simulink model "interleaved_boost"  (R2026b)
settings: Solver=ode23tb  StopTime=param.sim.simlength  FixedStep=tc  MaxStep=param.glb_time.tc
values from neighbouring files (symbols this model uses):
  param = struct()    [init_model.m]
libraries: fl_lib x138, nesl_utility x71, igbt_simple_2th_lib x6, single_phase_pwm_modulator x3, lithium_ion_battery x1, dclink_for_two_levels x1
(part 1 of 3)
settings Model: Creator=dbagn  LastModifiedBy=d.bagnara
settings SolverCC: SolverResetMethod=Robust  ZeroCrossControl=DisableAll
settings DataIOCC: DSMLogging=off  ReturnWorkspaceOutputs=off  SaveOutput=off  SaveTime=off  SignalLogging=off
settings OptimizationCC: ReuseModelBlockBuffer=off
settings SFSimCC: CustomCodeUndefinedFunction=ThrowError  DefaultCustomCodeDeterministicFunctions=All
settings SFSimCC: SimCustomHeaderCode=|
  | #include "rpi.h"
  | #include "rpi_simulink.h"
  | #include "bemf_obsv_load_est.h"
  | #include "bemf_obsv_load_est_simulink.h"
  | #include "dqpll_grid.h"
  | #include "dsmavgflt.h"
  | #include "bemf_obsv.h"
  | #include "bemf_obsv_simulink.h"
  | #include "mavgflt.h"
  | #include "mavgflt_simulink.h"
  | #include "mavgflts.h"
  | #include "mavgflts_simulink.h"
  | #include "sv_pwm_cm.h"
  | #include "dsmavgflt_simulink.h"
  | #include "linear_double_integrator_observer_simulink.h"
  | #include "sv_pwm_cm_simulink.h"
  | #include "dqvector_pi.h"
  | #include "dqpll_grid_simulink.h"
  | #include "first_harmonic_tracker.h"
  | #include "dqvector_pi_simulink.h"
  | #include "first_harmonic_tracker_simulink.h"
  | #include "dqpll_thyr.h"
  | #include "sv_pwm_simulink.h"
  | #include "sv_pwm.h"
  | #include "dqpll_thyr_simulink.h"
  | #include "linear_double_integrator_observer.h"
  | #include "math_f.h"
settings SFSimCC: SimUserIncludeDirs=|
  | include
  | src
settings SFSimCC: SimUserSources=|
  | "rpi.c"
  | "rpi_simulink.c"
  | "mavgflt_simulink.c"
  | "mavgflt.c"
  | "mavgflts_simulink.c"
  | "mavgflts.c"
  | "dsmavgflt_simulink.c"
  | "dsmavgflt.c"
  | "bemf_obsv_simulink.c"
  | "bemf_obsv.c"
  | "bemf_obsv_load_est_simulink.c"
  | "bemf_obsv_load_est.c"
  | "dqvector_pi.c"
  | "dqvector_pi_simulink.c"
  | "sv_pwm_simulink.c"
  | "sv_pwm.c"
  | "first_harmonic_tracker_simulink.c"
  | "first_harmonic_tracker.c"
  | "dqpll_thyr_simulink.c"
  | "dqpll_thyr.c"
  | "dqpll_grid_simulink.c"
  | "dqpll_grid.c"
  | "linear_double_integrator_observer_simulink.c"
  | "linear_double_integrator_observer.c"
  | "sv_pwm_cm_simulink.c"
  | "sv_pwm_cm.c"
settings RTWCC: DLArmComputeVersion=19.05
settings SimscapeCC: SimscapeUseEnergyAccounting=off

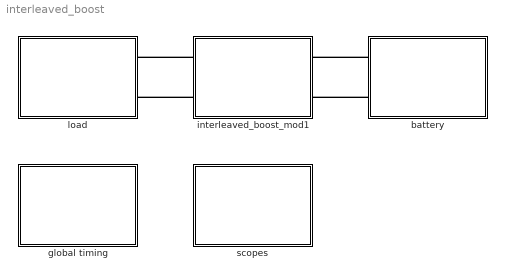
== system interleaved_boost ==
  battery : Subsystem
  global timing : Subsystem
  interleaved_boost_mod1 : Subsystem
  load : Subsystem
  scopes : Subsystem
  connections:
  interleaved_boost_mod1/RConn1 -- load/RConn1
  interleaved_boost_mod1/RConn2 -- load/RConn2
  battery/RConn2 -- interleaved_boost_mod1/LConn2
  battery/RConn1 -- interleaved_boost_mod1/LConn1

== system interleaved_boost/battery ==
  Electrical Reference : fl_lib/Electrical/Electrical Elements/Electrical Reference
  Solver Configuration : nesl_utility/Solver Configuration  PhysicalDomain=network_engine_domain  SubClassName=solver  LeftPortType=input  RightPortType=generic  Tones=[]  Harmonics=[]  SimulateNoise=off  Profile=off  UseLocalSampling=off  EnableSwitchedLinearOptims=on  FrequencyDomain=off  UseCCode=off  RelTol=0.001  AbsTol=0.001  MinStep=1e-09  ToWorkspace=off  RevertToSquareIcSolve=off  NumHomotopyIterations=100  PhasorMode=off  PhasorModeNumHarmonics=1  ConsistencySolver=NEWTON_XTOL_AFTER_FTOL  CanonicalOrdering=CANONICAL  OptimizeIntermediates=OPTIMIZED  MulticoreSolverChoice=BACKWARD_EULER  IndexReductionMethod=DerivativeReplacement  DoDC=on  ResidualTolerance=1e-09  ConsistencyTolSource=GLOBAL  ConsistencyAbsTol=0.001  ConsistencyRelTol=0.001  ConsistencyTolFactor=0.001  UseLocalSolver=on  LocalSolverChoice=NE_BACKWARD_EULER_ADVANCER  ResolveIndetEquations=on  FunctionEvalNumThread=1  LocalSolverSampleTime=param.glb_time.tc  DoFixedCost=on  MaxNonlinIter=param.sim.nonlinear_iterations  MaxModeIter=2  ComputeImpulses=off  ImpulseIterations=2  LinearAlgebra=auto  LinearAlgebraNumThread=0  EquationFormulation=NE_TIME_EF  DelaysMemoryBudget=1024  AutomaticFiltering=on  FilteringTimeConstant=0.001  PartitionStorageMethod=AS_NEEDED  PartitionMemoryBudget=1024  PartitionMethod=BALANCED  MultibodyUseLocalSolver=off  MultibodyLocalSolverChoice=ODE1  MultibodyLocalSolverSampleTime=0.001
  To Workspace14 : ToWorkspace  VariableName=battery_data  SampleTime=param.glb_time.tc
      settings: MaxDataPoints=param.glb_time.Nc  Decimation=param.glb_time.decimation_tc
  lithium-ion_battery : lithium_ion_battery/lithium_ion_battery  Q=param.battery.pack_1.Q  number_of_cells=param.battery.pack_1.number_of_cells  E_1=param.battery.pack_1.E_1  E0=param.battery.pack_1.E0  E1=param.battery.pack_1.E1  E2=param.battery.pack_1.E2  E3=param.battery.pack_1.E3  Elog=param.battery.pack_1.Elog  R0=param.battery.pack_1.R0  R1=param.battery.pack_1.R1  C1=param.battery.pack_1.C1  M=param.battery.pack_1.M  alpha=param.battery.pack_1.alpha  soc_init=param.battery.pack_1.soc_init  ts_battery=param.glb_time.ts_dab  q1Kalman=param.battery.pack_1.q1Kalman  q2Kalman=param.battery.pack_1.q2Kalman  q3Kalman=param.battery.pack_1.q3Kalman  rKalman=param.battery.pack_1.rKalman  tc=param.glb_time.tc  enable_white_noise_m=0  battery_voltage_init_m=param.battery.nominal_battery_voltage_1
  litium ion battery : Scope
      settings: ActiveDisplayYMinimum=703.3241597387879  ActiveDisplayYMaximum=878.06229440817833  DataLoggingVariableName=ScopeData3
  single_phase_ui_measure : Subsystem
  dc+ : PMIOPort  Side=Right
  dc- : PMIOPort  Port=2  Side=Right
  wires:
  lithium-ion_battery/1 -> To Workspace14/1, litium ion battery/1
  connections:
  lithium-ion_battery/RConn2 -- Solver Configuration/RConn1 -- Electrical Reference/LConn1 -- single_phase_ui_measure/LConn2
  single_phase_ui_measure/RConn1 -- dc+/RConn1
  lithium-ion_battery/RConn1 -- single_phase_ui_measure/LConn1
  dc-/RConn1 -- single_phase_ui_measure/RConn2

== system interleaved_boost/global timing ==
  Unit Delay : UnitDelay  SampleTime=param.glb_time.tc
  time_afe1 : Subsystem  mask{k=param.boost.behav.time_gain_module_1}
      mask prompts: k "Time Gain"
      mask Display:
      | disp('time-gen');
      | port_label('input', 1, 'crt');
      | port_label('output', 1, 'tout');
  time_afe3 : Subsystem  mask{k=1}
      mask prompts: k "Time Gain"
      mask Display:
      | disp('time-gen');
      | port_label('output', 1, 'tout');
  tag scope: time_afe_module_1=global, time_master=global
  wires:
  time_afe1/1(Out1) -> [time_afe_module_1]
  time_afe3/1(Out1) -> [time_master]
  [local_time_corr_afe1] -> Unit Delay/1
  Unit Delay/1 -> time_afe1/1(correction_time)

== system interleaved_boost/interleaved_boost_mod1 ==
  LRC_filter : Subsystem
  dcdc_ctrl : Subsystem
  interleaved_boost : Subsystem
  u_in(+) : PMIOPort  Side=Left
  u_in(-) : PMIOPort  Port=2  Side=Left
  Udc(+) : PMIOPort  Port=3  Side=Right
  Udc(-) : PMIOPort  Port=4  Side=Right
  wires:
  dcdc_ctrl/1(m_ctrl_out) -> interleaved_boost/1(dabc)
  connections:
  Udc(-)/RConn1 -- interleaved_boost/RConn2
  Udc(+)/RConn1 -- interleaved_boost/RConn1
  LRC_filter/LConn1 -- interleaved_boost/LConn1
  LRC_filter/LConn2 -- interleaved_boost/LConn2
  LRC_filter/LConn3 -- interleaved_boost/LConn3
  u_in(+)/RConn1 -- LRC_filter/RConn1
  u_in(-)/RConn1 -- LRC_filter/RConn2
  interleaved_boost/LConn4 -- LRC_filter/LConn4

== system interleaved_boost/load ==
  Resistor : fl_lib/Electrical/Electrical Elements/Resistor  R=param.load.R_load Ohm  i_specify=off  i_priority=None  i=0 A  i_nominal_specify=off  i_nominal_value=1  i_nominal_unit=A  v_specify=off  v_priority=None  v=0 V  v_nominal_specify=off  v_nominal_value=1  v_nominal_unit=V
  Udc(+) : PMIOPort  Side=Right
  Udc(-) : PMIOPort  Port=2  Side=Right
  connections:
  Resistor/LConn1 -- Udc(+)/RConn1
  Resistor/RConn1 -- Udc(-)/RConn1

== system interleaved_boost/scopes ==
  dcdc : Subsystem
  igbt_power_losses : Subsystem

== system interleaved_boost/battery/single_phase_ui_measure ==
  Bus Creator : BusCreator  Inputs=2
  Current Sensor : fl_lib/Electrical/Electrical Sensors/Current Sensor
  Selector : Selector  InputPortWidth=2  IndexOptions=Index vector (dialog)  Indices=2  OutputSizes=1  RuntimeRangeChecks=off
  Selector1 : Selector  InputPortWidth=2  IndexOptions=Index vector (dialog)  Indices=1  OutputSizes=1  RuntimeRangeChecks=off
  Voltage Sensor : fl_lib/Electrical/Electrical Sensors/Voltage Sensor
  dab input modA : Scope  NumInputPorts=2
      settings: SampleTime=param.glb_time.tc  ActiveDisplayYMinimum=-7186.64940163822  ActiveDisplayYMaximum=18834.744991863048  DataLoggingVariableName=ScopeData2
  iph : nesl_utility/PS-Simulink Converter  PhysicalDomain=network_engine_domain  SubClassName=ps_output  LeftPortType=input  RightPortType=output  PseudoPeriodic=off  Frequencies=[]  VectorFormat=1-D array  Unit=A  AffineConversion=off
  uph : nesl_utility/PS-Simulink Converter  PhysicalDomain=network_engine_domain  SubClassName=ps_output  LeftPortType=input  RightPortType=output  PseudoPeriodic=off  Frequencies=[]  VectorFormat=1-D array  Unit=V  AffineConversion=off
  Udc(+) : PMIOPort  Side=Left
  udc(+) : PMIOPort  Port=2  Side=Right
  Udc(-) : PMIOPort  Port=3  Side=Left
  udc(-) : PMIOPort  Port=4  Side=Right
  tag scope: current_battery=global, voltage_battery=global
  wires:
  Bus Creator/1 -> Selector/1, Selector1/1  "ui_data"
  iph/1 -> Bus Creator/1  "iph"
  uph/1 -> Bus Creator/2  "uph"
  Selector1/1 -> [current_battery], dab input modA/1  "current_battery"
  Selector/1 -> dab input modA/2, [voltage_battery]  "voltage_battery"
  connections:
  iph/LConn1 -- Current Sensor/RConn1
  Voltage Sensor/LConn1 -- Current Sensor/LConn1 -- Udc(+)/RConn1
  Current Sensor/RConn2 -- udc(+)/RConn1
  Voltage Sensor/RConn1 -- uph/LConn1
  Voltage Sensor/RConn2 -- Udc(-)/RConn1 -- udc(-)/RConn1

== system interleaved_boost/global timing/time_afe1 ==
  correction_time : Inport
  Constant : Constant
  Gain : Gain  Gain=k
  Product : Product
  Sum : Sum  Inputs=|++
  time_1 : Clock
  Out1 : Outport
  wires:
  time_1/1 -> Gain/1
  Gain/1 -> Product/1
  Product/1 -> Out1/1
  correction_time/1 -> Sum/1
  Sum/1 -> Product/2
  Constant/1 -> Sum/2

== system interleaved_boost/global timing/time_afe3 ==
  Gain : Gain  Gain=k
  time_1 : Clock
  Out1 : Outport
  wires:
  Gain/1 -> Out1/1
  time_1/1 -> Gain/1

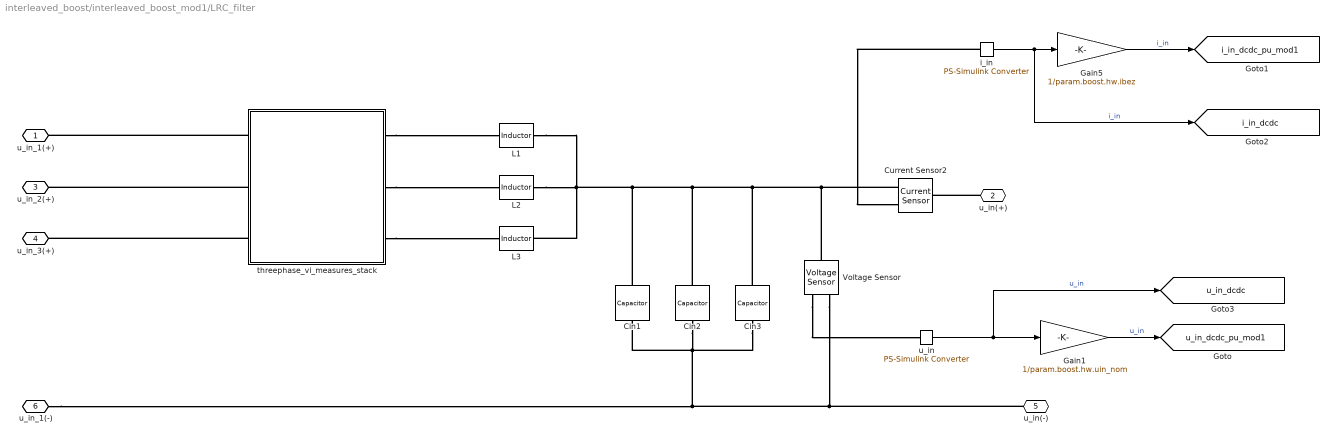
== system interleaved_boost/interleaved_boost_mod1/LRC_filter ==
  Cin1 : fl_lib/Electrical/Electrical Elements/Capacitor  c=param.boost.hw.Cin/3 F  r=3*param.boost.hw.RCin Ohm  g=0 1/Ohm  i_specify=off  i_priority=None  i=0 A  i_nominal_specify=off  i_nominal_value=1  i_nominal_unit=A  v_specify=off  v_priority=None  v=0 V  v_nominal_specify=off  v_nominal_value=1  v_nominal_unit=V  vc_specify=on  vc_priority=High  vc=param.boost.hw.Vin0 V  vc_nominal_specify=off  vc_nominal_value=1  vc_nominal_unit=V
  Cin2 : fl_lib/Electrical/Electrical Elements/Capacitor  c=param.boost.hw.Cin/3 F  r=3*param.boost.hw.RCin Ohm  g=0 1/Ohm  i_specify=off  i_priority=None  i=0 A  i_nominal_specify=off  i_nominal_value=1  i_nominal_unit=A  v_specify=off  v_priority=None  v=0 V  v_nominal_specify=off  v_nominal_value=1  v_nominal_unit=V  vc_specify=on  vc_priority=High  vc=param.boost.hw.Vin0 V  vc_nominal_specify=off  vc_nominal_value=1  vc_nominal_unit=V
  Cin3 : fl_lib/Electrical/Electrical Elements/Capacitor  c=param.boost.hw.Cin/3 F  r=3*param.boost.hw.RCin Ohm  g=0 1/Ohm  i_specify=off  i_priority=None  i=0 A  i_nominal_specify=off  i_nominal_value=1  i_nominal_unit=A  v_specify=off  v_priority=None  v=0 V  v_nominal_specify=off  v_nominal_value=1  v_nominal_unit=V  vc_specify=on  vc_priority=High  vc=param.boost.hw.Vin0 V  vc_nominal_specify=off  vc_nominal_value=1  vc_nominal_unit=V
  Current Sensor2 : fl_lib/Electrical/Electrical Sensors/Current Sensor
  Gain1 : Gain  Gain=1/param.boost.hw.uin_nom
  Gain5 : Gain  Gain=1/param.boost.hw.ibez
  L1 : fl_lib/Electrical/Electrical Elements/Inductor  l=param.boost.hw.L*param.boost.hw.kL(1) H  r=param.boost.hw.RL*param.boost.hw.kRL(1) Ohm  g=1e-9 1/Ohm  i_specify=on  i_priority=High  i=0 A  i_nominal_specify=off  i_nominal_value=1  i_nominal_unit=A  v_specify=off  v_priority=None  v=0 V  v_nominal_specify=off  v_nominal_value=1  v_nominal_unit=V  i_L_specify=off  i_L_priority=High  i_L=0 A  i_L_nominal_specify=off  i_L_nominal_value=1  i_L_nominal_unit=A
  L2 : fl_lib/Electrical/Electrical Elements/Inductor  l=param.boost.hw.L*param.boost.hw.kL(2) H  r=param.boost.hw.RL*param.boost.hw.kRL(2) Ohm  g=1e-9 1/Ohm  i_specify=on  i_priority=High  i=0 A  i_nominal_specify=off  i_nominal_value=1  i_nominal_unit=A  v_specify=off  v_priority=None  v=0 V  v_nominal_specify=off  v_nominal_value=1  v_nominal_unit=V  i_L_specify=off  i_L_priority=High  i_L=0 A  i_L_nominal_specify=off  i_L_nominal_value=1  i_L_nominal_unit=A
  L3 : fl_lib/Electrical/Electrical Elements/Inductor  l=param.boost.hw.L*param.boost.hw.kL(3) H  r=param.boost.hw.RL*param.boost.hw.kRL(3) Ohm  g=1e-9 1/Ohm  i_specify=on  i_priority=High  i=0 A  i_nominal_specify=off  i_nominal_value=1  i_nominal_unit=A  v_specify=off  v_priority=None  v=0 V  v_nominal_specify=off  v_nominal_value=1  v_nominal_unit=V  i_L_specify=off  i_L_priority=High  i_L=0 A  i_L_nominal_specify=off  i_L_nominal_value=1  i_L_nominal_unit=A
  Voltage Sensor : fl_lib/Electrical/Electrical Sensors/Voltage Sensor
  i_in : nesl_utility/PS-Simulink Converter  PhysicalDomain=network_engine_domain  SubClassName=ps_output  LeftPortType=input  RightPortType=output  PseudoPeriodic=off  Frequencies=[]  VectorFormat=1-D array  Unit=A  AffineConversion=off
  threephase_vi_measures_stack : Subsystem
  u_in : nesl_utility/PS-Simulink Converter  PhysicalDomain=network_engine_domain  SubClassName=ps_output  LeftPortType=input  RightPortType=output  PseudoPeriodic=off  Frequencies=[]  VectorFormat=1-D array  Unit=V  AffineConversion=off
  u_in_1(+) : PMIOPort  Side=Left
  u_in(+) : PMIOPort  Port=2  Side=Right
  u_in_2(+) : PMIOPort  Port=3  Side=Left
  u_in_3(+) : PMIOPort  Port=4  Side=Left
  u_in(-) : PMIOPort  Port=5  Side=Right
  u_in_1(-) : PMIOPort  Port=6  Side=Left
  tag scope: i_in_dcdc=global, i_in_dcdc_pu_mod1=global, u_in_dcdc=global, u_in_dcdc_pu_mod1=global
  wires:
  u_in/1 -> [u_in_dcdc], Gain1/1  "u_in"
  Gain1/1 -> [u_in_dcdc_pu_mod1]  "u_in"
  i_in/1 -> [i_in_dcdc], Gain5/1  "i_in"
  Gain5/1 -> [i_in_dcdc_pu_mod1]  "i_in"
  connections:
  Cin1/RConn1 -- Voltage Sensor/RConn2 -- u_in(-)/RConn1 -- u_in_1(-)/RConn1 -- Cin3/RConn1 -- Cin2/RConn1
  threephase_vi_measures_stack/LConn1 -- u_in_1(+)/RConn1
  threephase_vi_measures_stack/LConn2 -- u_in_2(+)/RConn1
  threephase_vi_measures_stack/LConn3 -- u_in_3(+)/RConn1
  L1/RConn1 -- Cin1/LConn1 -- Current Sensor2/RConn2 -- Voltage Sensor/LConn1 -- Cin3/LConn1 -- Cin2/LConn1 -- L3/RConn1 -- L2/RConn1
  Voltage Sensor/RConn1 -- u_in/LConn1
  i_in/LConn1 -- Current Sensor2/RConn1
  u_in(+)/RConn1 -- Current Sensor2/LConn1
  threephase_vi_measures_stack/RConn1 -- L1/LConn1
  threephase_vi_measures_stack/RConn2 -- L2/LConn1
  threephase_vi_measures_stack/RConn3 -- L3/LConn1

== system interleaved_boost/interleaved_boost_mod1/dcdc_ctrl ==
  boost_control : Subsystem
  is_hold : UnitDelay  SampleTime=param.glb_time.tc
  sample_hold_legs : Switch  Criteria=u2 > Threshold  Threshold=0.5  SaturateOnIntegerOverflow=off  InputSameDT=off
  trgo_leg1 : Selector  InputPortWidth=3  IndexOptions=Index vector (dialog)  Indices=1  OutputSizes=1  RuntimeRangeChecks=off
  m_ctrl_out : Outport
  wires:
  [u_in_dcdc_pu_mod1] -> boost_control/1(u_in_dcdc_pu)
  [vdc_pu_afe_mod1] -> boost_control/3(udc_pu)
  boost_control/1(m_ctrl_out) -> m_ctrl_out/1
  [i_in_dcdc_pu_mod1] -> boost_control/2(i_in_dcdc_pu)
  [TRGO_afe_module_1] -> sample_hold_legs/2, trgo_leg1/1
  trgo_leg1/1 -> boost_control/Trigger
  [is_abc_dcdc_pu_mod1] -> sample_hold_legs/1
  sample_hold_legs/1 -> boost_control/4(is_abc_dcdc_pu), is_hold/1
  is_hold/1 -> sample_hold_legs/3

== system interleaved_boost/interleaved_boost_mod1/interleaved_boost ==
  dabc : Inport
  Bus Selector : BusSelector  OutputSignals=vdc_pu
  Bus Selector1 : BusSelector  OutputSignals=udc,udc_p_gnd,udc_centertap_gnd,udc_n_gnd  OutputAsBus=on
  Bus Selector2 : BusSelector  OutputSignals=udc
  Bus Selector3 : BusSelector  OutputSignals=Cdc1_current
  dclink1 : dclink_for_two_levels/dclink  Cdc=param.boost.hw.Cdc  Rudc_measure=1e6  Vdc_scale=param.boost.hw.udc_nom
  three_phase_inverter_with_igbt_simple_2th : Subsystem
  tri-interleaved_boost_pwm : Subsystem
  Udc(+) : PMIOPort  Side=Right
  Udc(-) : PMIOPort  Port=2  Side=Right
  u_in_1(+) : PMIOPort  Port=3  Side=Left
  u_in_2(+) : PMIOPort  Port=4  Side=Left
  u_in_3(+) : PMIOPort  Port=5  Side=Left
  u_in(-) : PMIOPort  Port=6  Side=Left
  tag scope: all_voltages_about_dclink=global, ic_dclink_mod1=global, udc_mod1=global, vdc_pu_afe_mod1=global, vdc_pu_inv_mod1=global
  wires:
  dabc/1 -> tri-interleaved_boost_pwm/1(duties_uvw)
  tri-interleaved_boost_pwm/1(gate_cmds) -> three_phase_inverter_with_igbt_simple_2th/1(gate_commands)
  dclink1/1 -> Bus Selector1/1, Bus Selector2/1, Bus Selector3/1, Bus Selector/1
  Bus Selector1/1 -> [all_voltages_about_dclink]
  Bus Selector/1 -> [vdc_pu_afe_mod1], [vdc_pu_inv_mod1]  "<vdc_pu>"
  Bus Selector2/1 -> [udc_mod1]  "<udc>"
  Bus Selector3/1 -> [ic_dclink_mod1]  "<Cdc1_current>"
  connections:
  dclink1/RConn1 -- Udc(+)/RConn1
  dclink1/RConn2 -- Udc(-)/RConn1
  dclink1/LConn2 -- three_phase_inverter_with_igbt_simple_2th/LConn2
  dclink1/LConn1 -- three_phase_inverter_with_igbt_simple_2th/LConn1
  three_phase_inverter_with_igbt_simple_2th/RConn2 -- u_in_2(+)/RConn1
  three_phase_inverter_with_igbt_simple_2th/RConn3 -- u_in_3(+)/RConn1
  three_phase_inverter_with_igbt_simple_2th/RConn1 -- u_in_1(+)/RConn1
  u_in(-)/RConn1 -- three_phase_inverter_with_igbt_simple_2th/RConn4

== system interleaved_boost/scopes/dcdc ==
  Gain7 : Gain  Gain=param.boost.hw.ibez
  Gain8 : Gain  Gain=param.boost.hw.uin_nom
  i/u_in_dcdc : Scope  NumInputPorts=2
      settings: SampleTime=param.glb_time.tc  ActiveDisplayYMinimum=744.096505460461  ActiveDisplayYMaximum=804.97376748500153
  idc/udc : Scope  NumInputPorts=2
      settings: SampleTime=param.glb_time.tc  ActiveDisplayYMinimum=-239.04322132962466  ActiveDisplayYMaximum=376.33870683328587  DataLoggingVariableName=ScopeData23
  is/u_in_pu_mod1 : Scope  NumInputPorts=2
      settings: SampleTime=param.glb_time.tc  ActiveDisplayYMinimum=201.72238673067903  ActiveDisplayYMaximum=362.97459376282143  DataLoggingVariableName=ScopeData9
  udc voltages : Scope  NumInputPorts=2
      settings: SampleTime=param.glb_time.tc  ActiveDisplayYMinimum=0.94185811311147083  ActiveDisplayYMaximum=0.96255978130810615  DataLoggingVariableName=ScopeData24
  wires:
  [udc_mod1] -> idc/udc/2  "udc_dclink_mod1"
  Gain8/1 -> is/u_in_pu_mod1/2  "u_in_pu_mod1"
  [ic_dclink_mod1] -> idc/udc/1  "ic_dclink_mod1"
  [is_abc_dcdc_pu_mod1] -> Gain7/1
  [all_voltages_about_dclink] -> udc voltages/2  "all_voltages_about_dclink"
  Gain7/1 -> is/u_in_pu_mod1/1  "is_abc_pu_mod1"
  [u_in_dcdc_pu_mod1] -> Gain8/1
  [vdc_pu_afe_mod1] -> udc voltages/1  "udc"
  [u_in_dcdc] -> i/u_in_dcdc/2  "u_in_dcdc"
  [i_in_dcdc] -> i/u_in_dcdc/1  "i_in_dcdc"

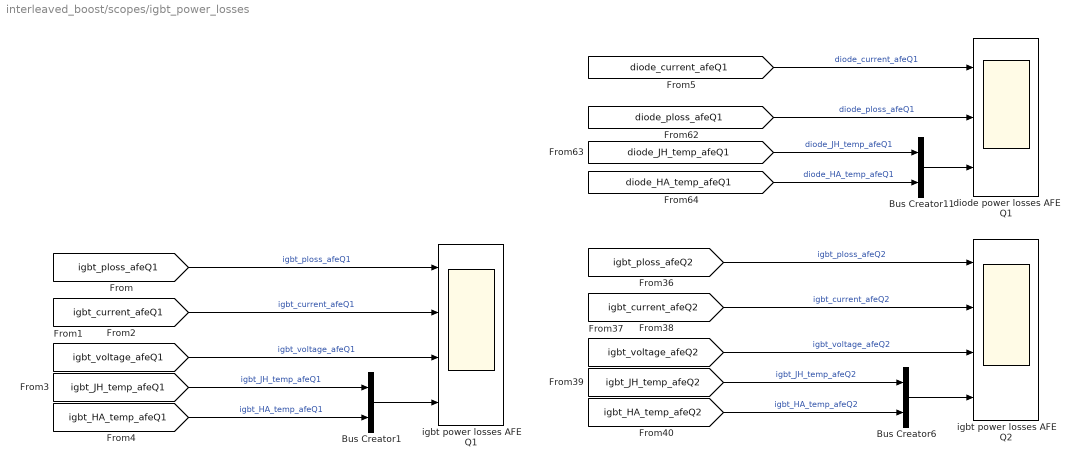
== system interleaved_boost/scopes/igbt_power_losses ==
  Bus Creator1 : BusCreator  Inputs=2
  Bus Creator11 : BusCreator  Inputs=2
  Bus Creator6 : BusCreator  Inputs=2
  diode power losses AFE Q1 : Scope  NumInputPorts=3
      settings: SampleTime=param.glb_time.tc  ActiveDisplayYMinimum=-5.1394924510579969  ActiveDisplayYMaximum=241.01139571693443  DataLoggingVariableName=ScopeData32
  igbt power losses AFE Q1 : Scope  NumInputPorts=4
      settings: SampleTime=param.glb_time.tc  ActiveDisplayYMinimum=-81.452854377977744  ActiveDisplayYMaximum=733.07569785592148  DataLoggingVariableName=ScopeData15
  igbt power losses AFE Q2 : Scope  NumInputPorts=4
      settings: SampleTime=param.glb_time.tc  ActiveDisplayYMinimum=-83.486123652533351  ActiveDisplayYMaximum=751.44374124171316  DataLoggingVariableName=ScopeData26
  wires:
  [igbt_ploss_afeQ1] -> igbt power losses AFE Q1/1  "igbt_ploss_afeQ1"
  [igbt_current_afeQ2] -> igbt power losses AFE Q2/2  "igbt_current_afeQ2"
  [igbt_ploss_afeQ2] -> igbt power losses AFE Q2/1  "igbt_ploss_afeQ2"
  [igbt_JH_temp_afeQ1] -> Bus Creator1/1  "igbt_JH_temp_afeQ1"
  [diode_JH_temp_afeQ1] -> Bus Creator11/1  "diode_JH_temp_afeQ1"
  [igbt_JH_temp_afeQ2] -> Bus Creator6/1  "igbt_JH_temp_afeQ2"
  Bus Creator11/1 -> diode power losses AFE Q1/3
  [igbt_HA_temp_afeQ2] -> Bus Creator6/2  "igbt_HA_temp_afeQ2"
  [diode_HA_temp_afeQ1] -> Bus Creator11/2  "diode_HA_temp_afeQ1"
  Bus Creator1/1 -> igbt power losses AFE Q1/4
  Bus Creator6/1 -> igbt power losses AFE Q2/4
  [igbt_voltage_afeQ1] -> igbt power losses AFE Q1/3  "igbt_voltage_afeQ1"
  [igbt_current_afeQ1] -> igbt power losses AFE Q1/2  "igbt_current_afeQ1"
  [igbt_HA_temp_afeQ1] -> Bus Creator1/2  "igbt_HA_temp_afeQ1"
  [diode_ploss_afeQ1] -> diode power losses AFE Q1/2  "diode_ploss_afeQ1"
  [igbt_voltage_afeQ2] -> igbt power losses AFE Q2/3  "igbt_voltage_afeQ2"
  [diode_current_afeQ1] -> diode power losses AFE Q1/1  "diode_current_afeQ1"

== system interleaved_boost/interleaved_boost_mod1/LRC_filter/threephase_vi_measures_stack ==
  Current Sensor : fl_lib/Electrical/Electrical Sensors/Current Sensor
  Current Sensor1 : fl_lib/Electrical/Electrical Sensors/Current Sensor
  Current Sensor2 : fl_lib/Electrical/Electrical Sensors/Current Sensor
  Gain4 : Gain  Gain=1/param.boost.hw.ibez
  Gain5 : Gain  Gain=1/param.boost.hw.ibez
  Gain6 : Gain  Gain=1/param.boost.hw.ibez
  ia_afe : nesl_utility/PS-Simulink Converter  PhysicalDomain=network_engine_domain  SubClassName=ps_output  LeftPortType=input  RightPortType=output  PseudoPeriodic=off  Frequencies=[]  VectorFormat=1-D array  Unit=A  AffineConversion=off
  ib_afe : nesl_utility/PS-Simulink Converter  PhysicalDomain=network_engine_domain  SubClassName=ps_output  LeftPortType=input  RightPortType=output  PseudoPeriodic=off  Frequencies=[]  VectorFormat=1-D array  Unit=A  AffineConversion=off
  ic_afe : nesl_utility/PS-Simulink Converter  PhysicalDomain=network_engine_domain  SubClassName=ps_output  LeftPortType=input  RightPortType=output  PseudoPeriodic=off  Frequencies=[]  VectorFormat=1-D array  Unit=A  AffineConversion=off
  is_legs_mux : Mux  Inputs=3
  Ua : PMIOPort  Side=Left
  ua : PMIOPort  Port=2  Side=Right
  Ub : PMIOPort  Port=3  Side=Left
  ub : PMIOPort  Port=4  Side=Right
  Uc : PMIOPort  Port=5  Side=Left
  uc : PMIOPort  Port=6  Side=Right
  tag scope: is_abc_dcdc_pu_mod1=global
  wires:
  is_legs_mux/1 -> [is_abc_dcdc_pu_mod1]
  ib_afe/1 -> Gain4/1  "ib_afe"
  ia_afe/1 -> Gain6/1  "ia_afe"
  ic_afe/1 -> Gain5/1  "ic_afe"
  Gain6/1 -> is_legs_mux/1  "ia_afe_pu"
  Gain4/1 -> is_legs_mux/2  "ib_afe_pu"
  Gain5/1 -> is_legs_mux/3  "ic_afe_pu"
  connections:
  Current Sensor1/RConn2 -- Ub/RConn1
  Current Sensor/LConn1 -- ua/RConn1
  Current Sensor2/RConn2 -- Uc/RConn1
  Current Sensor/RConn2 -- Ua/RConn1
  Current Sensor1/LConn1 -- ub/RConn1
  ib_afe/LConn1 -- Current Sensor1/RConn1
  ia_afe/LConn1 -- Current Sensor/RConn1
  ic_afe/LConn1 -- Current Sensor2/RConn1
  Current Sensor2/LConn1 -- uc/RConn1

== system interleaved_boost/interleaved_boost_mod1/dcdc_ctrl/boost_control ==
  u_in_dcdc_pu : Inport  PortDimensions=1
  i_in_dcdc_pu : Inport  Port=2  PortDimensions=1
  udc_pu : Inport  Port=3  PortDimensions=1
  is_abc_dcdc_pu : Inport  Port=4  PortDimensions=3
  Trigger : TriggerPort  VariantControl=(inherit)  PortDimensions=1
  Constant : Constant  Value=param.boost.ctrl.udc_ref
  Goto Tag Visibility : GotoTagVisibility  GotoTag=udc_d_pu
  Goto Tag Visibility1 : GotoTagVisibility  GotoTag=u_in_dcdc_pu_mod1
  Goto Tag Visibility2 : GotoTagVisibility  GotoTag=u_in_d_dcdc_pu
  Goto Tag Visibility3 : GotoTagVisibility  GotoTag=is_abc_d_dcdc_pu
  Goto Tag Visibility4 : GotoTagVisibility  GotoTag=i_in_d_dcdc_pu
  Terminator : Terminator
  acquisitions : Subsystem
  current_ctrl : Subsystem
  voltage_ctrl : Subsystem
  m_ctrl_out : Outport
  wires:
  current_ctrl/1(m_ctrl_out) -> m_ctrl_out/1
  u_in_dcdc_pu/1 -> acquisitions/1(u_in_dcdc_pu)
  udc_pu/1 -> acquisitions/2(udc_pu)
  is_abc_dcdc_pu/1 -> acquisitions/3(is_abc_dcdc_pu)
  Constant/1 -> voltage_ctrl/2(udc_ref)
  voltage_ctrl/1(i_ref) -> current_ctrl/1(i_ref)
  i_in_dcdc_pu/1 -> acquisitions/4(i_in_dcdc_pu)
  [udc_d_pu] -> voltage_ctrl/1(udc)
  [i_in_d_dcdc_pu] -> Terminator/1

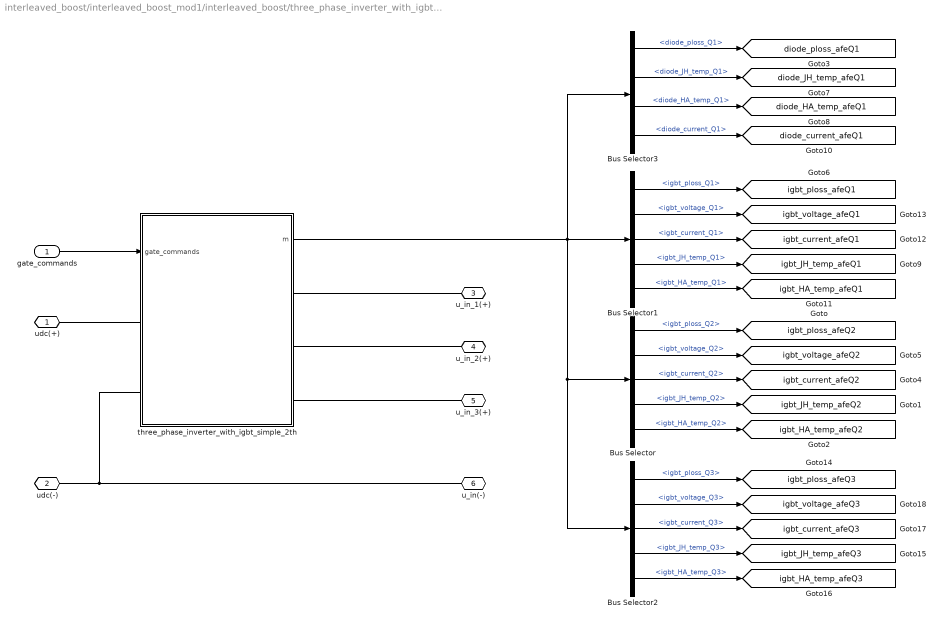
== system interleaved_boost/interleaved_boost_mod1/interleaved_boost/three_phase_inverter_with_igbt_simple_2th ==
  gate_commands : Inport
  Bus Selector : BusSelector  OutputSignals=module_1.igbt_ploss_Q2,module_1.igbt_voltage_Q2,module_1.igbt_current_Q2,module_1.igbt_JH_temp_Q2,module_1.igbt_HA_temp_Q2
  Bus Selector1 : BusSelector  OutputSignals=module_1.igbt_ploss_Q1,module_1.igbt_voltage_Q1,module_1.igbt_current_Q1,module_1.igbt_JH_temp_Q1,module_1.igbt_HA_temp_Q1
  Bus Selector2 : BusSelector  OutputSignals=module_2.igbt_ploss_Q3,module_2.igbt_voltage_Q3,module_2.igbt_current_Q3,module_2.igbt_JH_temp_Q3,module_2.igbt_HA_temp_Q3
  Bus Selector3 : BusSelector  OutputSignals=module_1.diode_ploss_Q1,module_1.diode_JH_temp_Q1,module_1.diode_HA_temp_Q1,module_1.diode_current_Q1
  three_phase_inverter_with_igbt_simple_2th : Subsystem  mask{vce_sat_m=param.boost.igbt.Vce_sat, v_gamma_m=param.boost.igbt.Vdon_diode, Vth_gate_m=param.boost.igbt.Vth, Vth_gate_hyst_m=0.85, Eon_m=param.boost.igbt.Eon*1000, Eoff_m=param.boost.igbt.Eoff*1000, Err_m=param.boost.igbt.Erec*1000, Ic_ref_m=param.boost.igbt.Ion_sw_losses, Vdc_ref_m=param.boost.igbt.Voff_sw_losses, Vblock_Errf_m=50, rce_on_m=param.boost.igbt.Rce_on*1000, rd_on_m=param.boost.igbt.Rdon_diode*1000, Gce_off_m=1e-6, time_constant_edge_m=param.glb_time.tc, time_constant_ploss_m=1e3, Csnubber_m=param.boost.igbt.Csnubber_zvs, Rsnubber_m=param.boost.igbt.Rsnubber_zvs, rth_switch_JH_m=param.boost.igbt.Rth_switch_JH, rth_switch_HA_m=param.thermal.heatsink.Rth_switch_HA, rth_diode_JH_m=param.boost.igbt.Rth_diode_JH, rth_diode_HA_m=param.thermal.heatsink.Rth_diode_HA, JunctionTermalMass_m=param.boost.igbt.JunctionTermalMass, Tambient_m=param.thermal.Tambient, mass_heatsink_m=param.thermal.heatsink.no_weight, specific_heat_m=param.thermal.heatsink.cp}
      mask prompts: vce_sat_m "Collector-emitter on-stage voltage [V]"; v_gamma_m "Diode forward voltage [V]"; Vth_gate_m "Gate-emitter threshold voltage [V]"; Vth_gate_hyst_m "Half hysteresis band for the switching events [V]"; Eon_m "Turn-on energy at Ic_ref, Vdc_ref [mJ]"; Eoff_m "Turn-off energy at Ic_ref, Vdc_ref [mJ]"; Err_m "Reverse recovery energy at Ic_ref, Vdc_ref [mJ]"; Ic_ref_m "Reference current of the energies [A]"; Vdc_ref_m "Reference voltage of the energies [V]"; Vblock_Errf_m "V block Err"; rce_on_m "IGBT on-state series resistance [mOhm]"; rd_on_m "Diode series resistance [mOhm]"; Gce_off_m "Off-state conductance [1/Ohm]"; time_constant_edge_m "Sample&hold time constant (<< on-time) [us]"; time_constant_ploss_m "Loss averaging time constant (2-5 x Tsw) [us]"; Csnubber_m "Csnubber [F]"; Rsnubber_m "Rsnubber [Ohm]"; rth_switch_JH_m "Thermal impedance Junction-heatsink switch [K/W]"; rth_switch_HA_m "Thermal impedance heatsink-ambient switch[K/W]"; rth_diode_JH_m "Thermal impedance Junction-heatsink diode [K/W]"; rth_diode_HA_m "Thermal impedance heatsink-ambient diode [K/W]"; JunctionTermalMass_m "Junction Thermal Mass [J/K]"; Tambient_m "Ambient temperature [degC]"; mass_heatsink_m "Mass heatsink [kg]"; specific_heat_m "Specific heat capacity of the heatsink [J/K/Kg]"
  udc(+) : PMIOPort  Side=Left
  udc(-) : PMIOPort  Port=2  Side=Left
  u_in_1(+) : PMIOPort  Port=3  Side=Right
  u_in_2(+) : PMIOPort  Port=4  Side=Right
  u_in_3(+) : PMIOPort  Port=5  Side=Right
  u_in(-) : PMIOPort  Port=6  Side=Right
  tag scope: diode_HA_temp_afeQ1=global, diode_JH_temp_afeQ1=global, diode_current_afeQ1=global, diode_ploss_afeQ1=global, igbt_HA_temp_afeQ1=global, igbt_HA_temp_afeQ2=global, igbt_HA_temp_afeQ3=global, igbt_JH_temp_afeQ1=global, igbt_JH_temp_afeQ2=global, igbt_JH_temp_afeQ3=global, igbt_current_afeQ1=global, igbt_current_afeQ2=global, igbt_current_afeQ3=global, igbt_ploss_afeQ1=global, igbt_ploss_afeQ2=global, igbt_ploss_afeQ3=global, igbt_voltage_afeQ1=global, igbt_voltage_afeQ2=global, igbt_voltage_afeQ3=global
  wires:
  gate_commands/1 -> three_phase_inverter_with_igbt_simple_2th/1(gate_commands)
  Bus Selector3/3 -> [diode_HA_temp_afeQ1]  "<diode_HA_temp_Q1>"
  Bus Selector/1 -> [igbt_ploss_afeQ2]  "<igbt_ploss_Q2>"
  Bus Selector3/2 -> [diode_JH_temp_afeQ1]  "<diode_JH_temp_Q1>"
  Bus Selector1/2 -> [igbt_voltage_afeQ1]  "<igbt_voltage_Q1>"
  Bus Selector/2 -> [igbt_voltage_afeQ2]  "<igbt_voltage_Q2>"
  Bus Selector/5 -> [igbt_HA_temp_afeQ2]  "<igbt_HA_temp_Q2>"
  Bus Selector2/5 -> [igbt_HA_temp_afeQ3]  "<igbt_HA_temp_Q3>"
  Bus Selector2/2 -> [igbt_voltage_afeQ3]  "<igbt_voltage_Q3>"
  Bus Selector/4 -> [igbt_JH_temp_afeQ2]  "<igbt_JH_temp_Q2>"
  Bus Selector1/4 -> [igbt_JH_temp_afeQ1]  "<igbt_JH_temp_Q1>"
  Bus Selector3/1 -> [diode_ploss_afeQ1]  "<diode_ploss_Q1>"
  Bus Selector2/4 -> [igbt_JH_temp_afeQ3]  "<igbt_JH_temp_Q3>"
  Bus Selector2/3 -> [igbt_current_afeQ3]  "<igbt_current_Q3>"
  three_phase_inverter_with_igbt_simple_2th/1(m) -> Bus Selector3/1, Bus Selector2/1, Bus Selector/1, Bus Selector1/1
  Bus Selector1/3 -> [igbt_current_afeQ1]  "<igbt_current_Q1>"
  Bus Selector/3 -> [igbt_current_afeQ2]  "<igbt_current_Q2>"
  Bus Selector1/5 -> [igbt_HA_temp_afeQ1]  "<igbt_HA_temp_Q1>"
  Bus Selector2/1 -> [igbt_ploss_afeQ3]  "<igbt_ploss_Q3>"
  Bus Selector1/1 -> [igbt_ploss_afeQ1]  "<igbt_ploss_Q1>"
  Bus Selector3/4 -> [diode_current_afeQ1]  "<diode_current_Q1>"
  connections:
  u_in_1(+)/RConn1 -- three_phase_inverter_with_igbt_simple_2th/RConn1
  udc(-)/RConn1 -- u_in(-)/RConn1 -- three_phase_inverter_with_igbt_simple_2th/LConn2
  udc(+)/RConn1 -- three_phase_inverter_with_igbt_simple_2th/LConn1
  three_phase_inverter_with_igbt_simple_2th/RConn2 -- u_in_2(+)/RConn1
  three_phase_inverter_with_igbt_simple_2th/RConn3 -- u_in_3(+)/RConn1

== system interleaved_boost/interleaved_boost_mod1/interleaved_boost/tri-interleaved_boost_pwm ==
  duties_uvw : Inport  PortDimensions=3
  Demux : Demux  Outputs=3
  Mux : Mux  Inputs=3
  td2tc_1 : TransferFcn  Denominator=[param.glb_time.tc 1]
  td2tc_2 : TransferFcn  Denominator=[param.glb_time.tc 1]
  td2tc_3 : TransferFcn  Denominator=[param.glb_time.tc 1]
  tri-interleaved_legs_modulator : Subsystem
  gate_cmds : Outport
  wires:
  tri-interleaved_legs_modulator/1(gate_cmds) -> gate_cmds/1
  duties_uvw/1 -> Demux/1
  Demux/1 -> td2tc_1/1
  Demux/2 -> td2tc_2/1
  Demux/3 -> td2tc_3/1
  td2tc_1/1 -> Mux/1
  td2tc_2/1 -> Mux/2
  td2tc_3/1 -> Mux/3
  Mux/1 -> tri-interleaved_legs_modulator/1(m)

== system interleaved_boost/interleaved_boost_mod1/dcdc_ctrl/boost_control/acquisitions ==
  u_in_dcdc_pu : Inport  PortDimensions=1
  udc_pu : Inport  Port=2  PortDimensions=1
  is_abc_dcdc_pu : Inport  Port=3  PortDimensions=3
  i_in_dcdc_pu : Inport  Port=4  PortDimensions=1
  Terminator : Terminator
  quantizzation and one step delay 1 : Subsystem
  quantizzation and one step delay 2 : Subsystem
  quantizzation and one step delay 3 : Subsystem
  udc_acquisition : Subsystem
  tag scope: i_in_d_dcdc_pu=scoped, is_abc_d_dcdc_pu=scoped, u_in_d_dcdc_pu=scoped, udc_d_pu=scoped
  wires:
  udc_acquisition/1(udcd_pu) -> [udc_d_pu]
  u_in_dcdc_pu/1 -> quantizzation and one step delay 1/1(u_in_dcdc_pu)
  [udc_d_pu] -> Terminator/1
  is_abc_dcdc_pu/1 -> quantizzation and one step delay 2/1(is_abc_dcdc_pu)
  udc_pu/1 -> udc_acquisition/1(udc_pu)
  quantizzation and one step delay 2/1(is_abc_d_dcdc_pu) -> [is_abc_d_dcdc_pu]
  quantizzation and one step delay 1/1(u_in_d_dcdc_pu) -> [u_in_d_dcdc_pu]
  i_in_dcdc_pu/1 -> quantizzation and one step delay 3/1(i_in_dcdc_pu)
  quantizzation and one step delay 3/1(i_in_d_dcdc_pu) -> [i_in_d_dcdc_pu]

== system interleaved_boost/interleaved_boost_mod1/dcdc_ctrl/boost_control/current_ctrl ==
  i_ref : Inport  PortDimensions=1
  one : Constant
  one_minus_d : Sum  Inputs=+-
  per_leg_ref : Gain  Gain=1/param.boost.hw.n_legs
  pi : Subsystem
  m_ctrl_out : Outport  VectorParamsAs1DForOutWhenUnconnected=off
  wires:
  pi/1(d_ctrl_out) -> one_minus_d/2
  one/1 -> one_minus_d/1
  one_minus_d/1 -> m_ctrl_out/1
  i_ref/1 -> per_leg_ref/1
  per_leg_ref/1 -> pi/2(id_ref)
  [is_abc_d_dcdc_pu] -> pi/1(id)  "i_legs"

== system interleaved_boost/interleaved_boost_mod1/dcdc_ctrl/boost_control/voltage_ctrl ==
  udc : Inport  PortDimensions=1
  udc_ref : Inport  Port=2  PortDimensions=1
  Sum1 : Sum  Inputs=|-+
  i_ref_limit : Saturate  UpperLimit=param.boost.ctrl.i_lim  LowerLimit=-param.boost.ctrl.i_lim
  pi_u : Subsystem
  ramp_limit : MinMax  Inputs=2
  ramp_state : UnitDelay  InitialCondition=param.boost.ctrl.udc_ref_init  SampleTime=-1
  ramp_step : Constant  Value=param.boost.ctrl.u_ref_slew*param.glb_time.ts_afe
  ramp_sum : Sum
  udc/udc_ref : Scope  NumInputPorts=2
      settings: ActiveDisplayYMinimum=0.94307980299057792  ActiveDisplayYMaximum=1.0559111812257966
  i_ref : Outport
  wires:
  Sum1/1 -> pi_u/1(id_tilde)
  udc/1 -> udc/udc_ref/1, Sum1/1  "udc"
  udc_ref/1 -> ramp_limit/2  "udc_ref"
  ramp_step/1 -> ramp_sum/1
  ramp_state/1 -> ramp_sum/2
  ramp_sum/1 -> ramp_limit/1
  ramp_limit/1 -> Sum1/2, ramp_state/1, udc/udc_ref/2
  pi_u/1(ud_out) -> i_ref_limit/1
  i_ref_limit/1 -> i_ref/1

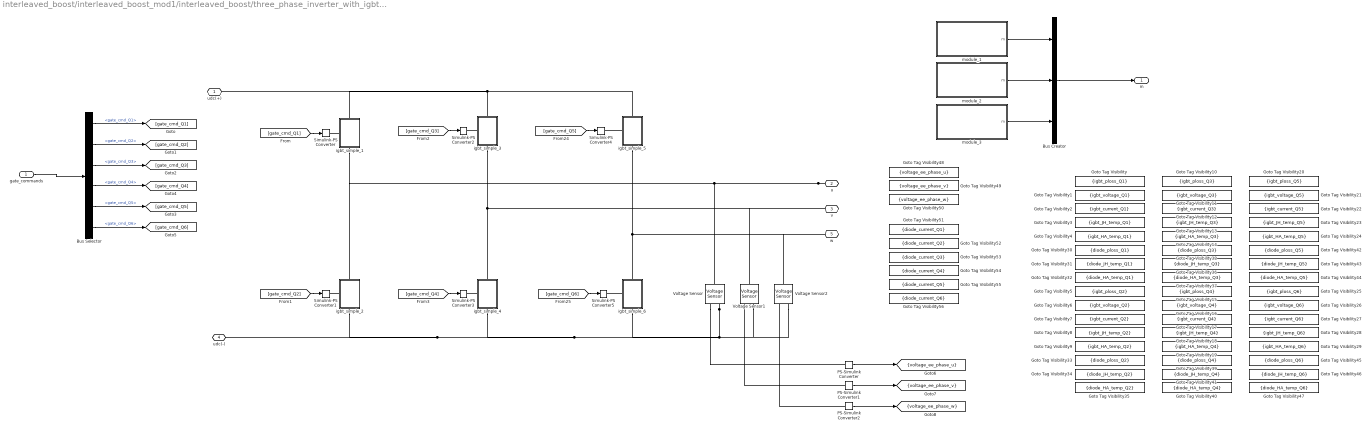
== system interleaved_boost/interleaved_boost_mod1/interleaved_boost/three_phase_inverter_with_igbt_simple_2th/three_phase_inverter_with_igbt_simple_2th ==
  gate_commands : Inport
  Bus Creator : BusCreator  Inputs=3
  Bus Selector : BusSelector  OutputSignals=signal1.gate_cmd_Q1,signal1.gate_cmd_Q2,signal2.gate_cmd_Q3,signal2.gate_cmd_Q4,signal3.gate_cmd_Q5,signal3.gate_cmd_Q6
  Goto Tag Visibility : GotoTagVisibility  GotoTag=igbt_ploss_Q1
  Goto Tag Visibility1 : GotoTagVisibility  GotoTag=igbt_voltage_Q1
  Goto Tag Visibility10 : GotoTagVisibility  GotoTag=igbt_ploss_Q3
  Goto Tag Visibility11 : GotoTagVisibility  GotoTag=igbt_voltage_Q3
  Goto Tag Visibility12 : GotoTagVisibility  GotoTag=igbt_current_Q3
  Goto Tag Visibility13 : GotoTagVisibility  GotoTag=igbt_JH_temp_Q3
  Goto Tag Visibility14 : GotoTagVisibility  GotoTag=igbt_HA_temp_Q3
  Goto Tag Visibility15 : GotoTagVisibility  GotoTag=igbt_ploss_Q4
  Goto Tag Visibility16 : GotoTagVisibility  GotoTag=igbt_voltage_Q4
  Goto Tag Visibility17 : GotoTagVisibility  GotoTag=igbt_current_Q4
  Goto Tag Visibility18 : GotoTagVisibility  GotoTag=igbt_JH_temp_Q4
  Goto Tag Visibility19 : GotoTagVisibility  GotoTag=igbt_HA_temp_Q4
  Goto Tag Visibility2 : GotoTagVisibility  GotoTag=igbt_current_Q1
  Goto Tag Visibility20 : GotoTagVisibility  GotoTag=igbt_ploss_Q5
  Goto Tag Visibility21 : GotoTagVisibility  GotoTag=igbt_voltage_Q5
  Goto Tag Visibility22 : GotoTagVisibility  GotoTag=igbt_current_Q5
  Goto Tag Visibility23 : GotoTagVisibility  GotoTag=igbt_JH_temp_Q5
  Goto Tag Visibility24 : GotoTagVisibility  GotoTag=igbt_HA_temp_Q5
  Goto Tag Visibility25 : GotoTagVisibility  GotoTag=igbt_ploss_Q6
  Goto Tag Visibility26 : GotoTagVisibility  GotoTag=igbt_voltage_Q6
  Goto Tag Visibility27 : GotoTagVisibility  GotoTag=igbt_current_Q6
  Goto Tag Visibility28 : GotoTagVisibility  GotoTag=igbt_JH_temp_Q6
  Goto Tag Visibility29 : GotoTagVisibility  GotoTag=igbt_HA_temp_Q6
  Goto Tag Visibility3 : GotoTagVisibility  GotoTag=igbt_JH_temp_Q1
  Goto Tag Visibility30 : GotoTagVisibility  GotoTag=diode_ploss_Q1
  Goto Tag Visibility31 : GotoTagVisibility  GotoTag=diode_JH_temp_Q1
  Goto Tag Visibility32 : GotoTagVisibility  GotoTag=diode_HA_temp_Q1
  Goto Tag Visibility33 : GotoTagVisibility  GotoTag=diode_ploss_Q2
  Goto Tag Visibility34 : GotoTagVisibility  GotoTag=diode_JH_temp_Q2
  Goto Tag Visibility35 : GotoTagVisibility  GotoTag=diode_HA_temp_Q2
  Goto Tag Visibility36 : GotoTagVisibility  GotoTag=diode_JH_temp_Q3
  Goto Tag Visibility37 : GotoTagVisibility  GotoTag=diode_HA_temp_Q3
  Goto Tag Visibility38 : GotoTagVisibility  GotoTag=diode_ploss_Q3
  Goto Tag Visibility39 : GotoTagVisibility  GotoTag=diode_ploss_Q4
  Goto Tag Visibility4 : GotoTagVisibility  GotoTag=igbt_HA_temp_Q1
  Goto Tag Visibility40 : GotoTagVisibility  GotoTag=diode_HA_temp_Q4
  Goto Tag Visibility41 : GotoTagVisibility  GotoTag=diode_JH_temp_Q4
  Goto Tag Visibility42 : GotoTagVisibility  GotoTag=diode_ploss_Q5
  Goto Tag Visibility43 : GotoTagVisibility  GotoTag=diode_JH_temp_Q5
  Goto Tag Visibility44 : GotoTagVisibility  GotoTag=diode_HA_temp_Q5
  Goto Tag Visibility45 : GotoTagVisibility  GotoTag=diode_ploss_Q6
  Goto Tag Visibility46 : GotoTagVisibility  GotoTag=diode_JH_temp_Q6
  Goto Tag Visibility47 : GotoTagVisibility  GotoTag=diode_HA_temp_Q6
  Goto Tag Visibility48 : GotoTagVisibility  GotoTag=voltage_ee_phase_u
  Goto Tag Visibility49 : GotoTagVisibility  GotoTag=voltage_ee_phase_v
  Goto Tag Visibility5 : GotoTagVisibility  GotoTag=igbt_ploss_Q2
  Goto Tag Visibility50 : GotoTagVisibility  GotoTag=voltage_ee_phase_w
  Goto Tag Visibility51 : GotoTagVisibility  GotoTag=diode_current_Q1
  Goto Tag Visibility52 : GotoTagVisibility  GotoTag=diode_current_Q2
  Goto Tag Visibility53 : GotoTagVisibility  GotoTag=diode_current_Q3
  Goto Tag Visibility54 : GotoTagVisibility  GotoTag=diode_current_Q4
  Goto Tag Visibility55 : GotoTagVisibility  GotoTag=diode_current_Q5
  Goto Tag Visibility56 : GotoTagVisibility  GotoTag=diode_current_Q6
  Goto Tag Visibility6 : GotoTagVisibility  GotoTag=igbt_voltage_Q2
  Goto Tag Visibility7 : GotoTagVisibility  GotoTag=igbt_current_Q2
  Goto Tag Visibility8 : GotoTagVisibility  GotoTag=igbt_JH_temp_Q2
  Goto Tag Visibility9 : GotoTagVisibility  GotoTag=igbt_HA_temp_Q2
  PS-Simulink Converter : nesl_utility/PS-Simulink Converter  PhysicalDomain=network_engine_domain  SubClassName=ps_output  LeftPortType=input  RightPortType=output  PseudoPeriodic=off  Frequencies=[]  VectorFormat=1-D array  Unit=V  AffineConversion=off
  PS-Simulink Converter1 : nesl_utility/PS-Simulink Converter  PhysicalDomain=network_engine_domain  SubClassName=ps_output  LeftPortType=input  RightPortType=output  PseudoPeriodic=off  Frequencies=[]  VectorFormat=1-D array  Unit=V  AffineConversion=off
  PS-Simulink Converter2 : nesl_utility/PS-Simulink Converter  PhysicalDomain=network_engine_domain  SubClassName=ps_output  LeftPortType=input  RightPortType=output  PseudoPeriodic=off  Frequencies=[]  VectorFormat=1-D array  Unit=V  AffineConversion=off
  Simulink-PS Converter{,1..5} (6 alike) : nesl_utility/Simulink-PS Converter  PhysicalDomain=network_engine_domain  SubClassName=ps_input  LeftPortType=input  RightPortType=output  PseudoPeriodic=off  Frequencies=[]  NoiseDistribution=none  NoiseParameters=[]  Unit=V  AffineConversion=off  FilteringAndDerivatives=provide  SimscapeFilterOrder=1  InputFilterTimeConstant=0.001  UdotUserProvided=0
  Voltage Sensor : fl_lib/Electrical/Electrical Sensors/Voltage Sensor
  Voltage Sensor1 : fl_lib/Electrical/Electrical Sensors/Voltage Sensor
  Voltage Sensor2 : fl_lib/Electrical/Electrical Sensors/Voltage Sensor
  igbt_simple_1 : Subsystem
      settings: PortSchema="{\"entries\":[{\"content\":{\"sides\":[{\"content\":{\"connectorIds\":[\"LConn1\"]},\"type\":\"ConnectorPlacement.EquallySpacedRectSide\",\"uuid\":\"9277da8d-d460-43e6-8478-dd662f15d226\"},{\"content\":{\"connectorIds\":[],\"side\":\"RIGHT\"},\"type\":\"ConnectorPlacement.EquallySpacedRectSide\",\"uuid\":\"a7ece396-f1d9-4f4f-a05b-db1fc65d6e1d\"},{\"content\":{\"connectorIds\":[\"LConn2\"],\"side\":\"TOP\"},\"type\":\"ConnectorPlacement.EquallySpacedRectSide\",\"uuid\":\"fdd70777-e9cf-4317-afb6-cae87f75d5b0\"},{\"content\":{\"connectorIds\":[\"RConn1\"],\"side\":\"BOTTOM\"},\"type\":\"ConnectorPlacement.EquallySpacedRectSide\",\"uuid\":\"2353ed68-b1a1-4775-9ca9-31e268d5443b\"}]},\"type\":\"ConnectorPlacement.EquallySpacedConnector\",\"uuid\":\"d5479f4c-4e65-4791-adcb-73df11f88590\"}],\"packageUris\":[\"http://schema.mathworks.com/mf0/Connector/R2020b\"],\"version\":\"1.0\"}"
  igbt_simple_2 : Subsystem
      settings: PortSchema="{\"entries\":[{\"content\":{\"sides\":[{\"content\":{\"connectorIds\":[\"LConn1\"]},\"type\":\"ConnectorPlacement.EquallySpacedRectSide\",\"uuid\":\"9277da8d-d460-43e6-8478-dd662f15d226\"},{\"content\":{\"connectorIds\":[],\"side\":\"RIGHT\"},\"type\":\"ConnectorPlacement.EquallySpacedRectSide\",\"uuid\":\"a7ece396-f1d9-4f4f-a05b-db1fc65d6e1d\"},{\"content\":{\"connectorIds\":[\"LConn2\"],\"side\":\"TOP\"},\"type\":\"ConnectorPlacement.EquallySpacedRectSide\",\"uuid\":\"fdd70777-e9cf-4317-afb6-cae87f75d5b0\"},{\"content\":{\"connectorIds\":[\"RConn1\"],\"side\":\"BOTTOM\"},\"type\":\"ConnectorPlacement.EquallySpacedRectSide\",\"uuid\":\"2353ed68-b1a1-4775-9ca9-31e268d5443b\"}]},\"type\":\"ConnectorPlacement.EquallySpacedConnector\",\"uuid\":\"d5479f4c-4e65-4791-adcb-73df11f88590\"}],\"packageUris\":[\"http://schema.mathworks.com/mf0/Connector/R2020b\"],\"version\":\"1.0\"}"
  igbt_simple_3 : Subsystem
      settings: PortSchema="{\"entries\":[{\"content\":{\"sides\":[{\"content\":{\"connectorIds\":[\"LConn1\"]},\"type\":\"ConnectorPlacement.EquallySpacedRectSide\",\"uuid\":\"9277da8d-d460-43e6-8478-dd662f15d226\"},{\"content\":{\"connectorIds\":[],\"side\":\"RIGHT\"},\"type\":\"ConnectorPlacement.EquallySpacedRectSide\",\"uuid\":\"a7ece396-f1d9-4f4f-a05b-db1fc65d6e1d\"},{\"content\":{\"connectorIds\":[\"LConn2\"],\"side\":\"TOP\"},\"type\":\"ConnectorPlacement.EquallySpacedRectSide\",\"uuid\":\"fdd70777-e9cf-4317-afb6-cae87f75d5b0\"},{\"content\":{\"connectorIds\":[\"RConn1\"],\"side\":\"BOTTOM\"},\"type\":\"ConnectorPlacement.EquallySpacedRectSide\",\"uuid\":\"2353ed68-b1a1-4775-9ca9-31e268d5443b\"}]},\"type\":\"ConnectorPlacement.EquallySpacedConnector\",\"uuid\":\"d5479f4c-4e65-4791-adcb-73df11f88590\"}],\"packageUris\":[\"http://schema.mathworks.com/mf0/Connector/R2020b\"],\"version\":\"1.0\"}"
  igbt_simple_4 : Subsystem
      settings: PortSchema="{\"entries\":[{\"content\":{\"sides\":[{\"content\":{\"connectorIds\":[\"LConn1\"]},\"type\":\"ConnectorPlacement.EquallySpacedRectSide\",\"uuid\":\"9277da8d-d460-43e6-8478-dd662f15d226\"},{\"content\":{\"connectorIds\":[],\"side\":\"RIGHT\"},\"type\":\"ConnectorPlacement.EquallySpacedRectSide\",\"uuid\":\"a7ece396-f1d9-4f4f-a05b-db1fc65d6e1d\"},{\"content\":{\"connectorIds\":[\"LConn2\"],\"side\":\"TOP\"},\"type\":\"ConnectorPlacement.EquallySpacedRectSide\",\"uuid\":\"fdd70777-e9cf-4317-afb6-cae87f75d5b0\"},{\"content\":{\"connectorIds\":[\"RConn1\"],\"side\":\"BOTTOM\"},\"type\":\"ConnectorPlacement.EquallySpacedRectSide\",\"uuid\":\"2353ed68-b1a1-4775-9ca9-31e268d5443b\"}]},\"type\":\"ConnectorPlacement.EquallySpacedConnector\",\"uuid\":\"d5479f4c-4e65-4791-adcb-73df11f88590\"}],\"packageUris\":[\"http://schema.mathworks.com/mf0/Connector/R2020b\"],\"version\":\"1.0\"}"
  igbt_simple_5 : Subsystem
      settings: PortSchema="{\"entries\":[{\"content\":{\"sides\":[{\"content\":{\"connectorIds\":[\"LConn1\"]},\"type\":\"ConnectorPlacement.EquallySpacedRectSide\",\"uuid\":\"9277da8d-d460-43e6-8478-dd662f15d226\"},{\"content\":{\"connectorIds\":[],\"side\":\"RIGHT\"},\"type\":\"ConnectorPlacement.EquallySpacedRectSide\",\"uuid\":\"a7ece396-f1d9-4f4f-a05b-db1fc65d6e1d\"},{\"content\":{\"connectorIds\":[\"LConn2\"],\"side\":\"TOP\"},\"type\":\"ConnectorPlacement.EquallySpacedRectSide\",\"uuid\":\"fdd70777-e9cf-4317-afb6-cae87f75d5b0\"},{\"content\":{\"connectorIds\":[\"RConn1\"],\"side\":\"BOTTOM\"},\"type\":\"ConnectorPlacement.EquallySpacedRectSide\",\"uuid\":\"2353ed68-b1a1-4775-9ca9-31e268d5443b\"}]},\"type\":\"ConnectorPlacement.EquallySpacedConnector\",\"uuid\":\"d5479f4c-4e65-4791-adcb-73df11f88590\"}],\"packageUris\":[\"http://schema.mathworks.com/mf0/Connector/R2020b\"],\"version\":\"1.0\"}"
  igbt_simple_6 : Subsystem
      settings: PortSchema="{\"entries\":[{\"content\":{\"sides\":[{\"content\":{\"connectorIds\":[\"LConn1\"]},\"type\":\"ConnectorPlacement.EquallySpacedRectSide\",\"uuid\":\"9277da8d-d460-43e6-8478-dd662f15d226\"},{\"content\":{\"connectorIds\":[],\"side\":\"RIGHT\"},\"type\":\"ConnectorPlacement.EquallySpacedRectSide\",\"uuid\":\"a7ece396-f1d9-4f4f-a05b-db1fc65d6e1d\"},{\"content\":{\"connectorIds\":[\"LConn2\"],\"side\":\"TOP\"},\"type\":\"ConnectorPlacement.EquallySpacedRectSide\",\"uuid\":\"fdd70777-e9cf-4317-afb6-cae87f75d5b0\"},{\"content\":{\"connectorIds\":[\"RConn1\"],\"side\":\"BOTTOM\"},\"type\":\"ConnectorPlacement.EquallySpacedRectSide\",\"uuid\":\"2353ed68-b1a1-4775-9ca9-31e268d5443b\"}]},\"type\":\"ConnectorPlacement.EquallySpacedConnector\",\"uuid\":\"d5479f4c-4e65-4791-adcb-73df11f88590\"}],\"packageUris\":[\"http://schema.mathworks.com/mf0/Connector/R2020b\"],\"version\":\"1.0\"}"
  module_1 : Subsystem
  module_2 : Subsystem
  module_3 : Subsystem
  udc(+) : PMIOPort  Side=Left
  u : PMIOPort  Port=2  Side=Right
  v : PMIOPort  Port=3  Side=Right
  udc(-) : PMIOPort  Port=4  Side=Left
  w : PMIOPort  Port=5  Side=Right
  m : Outport
  tag scope: voltage_ee_phase_u=scoped, voltage_ee_phase_v=scoped, voltage_ee_phase_w=scoped
  wires:
  module_3/1(m) -> Bus Creator/3
  module_1/1(m) -> Bus Creator/1
  Bus Creator/1 -> m/1
  module_2/1(m) -> Bus Creator/2
  PS-Simulink Converter2/1 -> [voltage_ee_phase_w]
  PS-Simulink Converter1/1 -> [voltage_ee_phase_v]
  PS-Simulink Converter/1 -> [voltage_ee_phase_u]
  [gate_cmd_Q6] -> Simulink-PS Converter5/1
  [gate_cmd_Q5] -> Simulink-PS Converter4/1
  [gate_cmd_Q3] -> Simulink-PS Converter2/1
  [gate_cmd_Q4] -> Simulink-PS Converter3/1
  [gate_cmd_Q2] -> Simulink-PS Converter1/1
  [gate_cmd_Q1] -> Simulink-PS Converter/1
  gate_commands/1 -> Bus Selector/1
  Bus Selector/6 -> [gate_cmd_Q6]  "<gate_cmd_Q6>"
  Bus Selector/5 -> [gate_cmd_Q5]  "<gate_cmd_Q5>"
  Bus Selector/4 -> [gate_cmd_Q4]  "<gate_cmd_Q4>"
  Bus Selector/3 -> [gate_cmd_Q3]  "<gate_cmd_Q3>"
  Bus Selector/2 -> [gate_cmd_Q2]  "<gate_cmd_Q2>"
  Bus Selector/1 -> [gate_cmd_Q1]  "<gate_cmd_Q1>"
  connections:
  PS-Simulink Converter2/LConn1 -- Voltage Sensor2/RConn1
  PS-Simulink Converter1/LConn1 -- Voltage Sensor1/RConn1
  Voltage Sensor/RConn1 -- PS-Simulink Converter/LConn1
  w/RConn1 -- Voltage Sensor2/LConn1 -- igbt_simple_6/LConn2 -- igbt_simple_5/RConn1
  v/RConn1 -- Voltage Sensor1/LConn1 -- igbt_simple_4/LConn2 -- igbt_simple_3/RConn1
  Voltage Sensor/RConn2 -- Voltage Sensor1/RConn2 -- Voltage Sensor2/RConn2 -- igbt_simple_6/RConn1 -- igbt_simple_4/RConn1 -- igbt_simple_2/RConn1 -- udc(-)/RConn1
  igbt_simple_6/LConn1 -- Simulink-PS Converter5/RConn1
  igbt_simple_5/LConn1 -- Simulink-PS Converter4/RConn1
  igbt_simple_4/LConn1 -- Simulink-PS Converter3/RConn1
  igbt_simple_3/LConn1 -- Simulink-PS Converter2/RConn1
  igbt_simple_2/LConn1 -- Simulink-PS Converter1/RConn1
  igbt_simple_1/LConn1 -- Simulink-PS Converter/RConn1
  udc(+)/RConn1 -- igbt_simple_1/LConn2 -- igbt_simple_5/LConn2 -- igbt_simple_3/LConn2
  u/RConn1 -- Voltage Sensor/LConn1 -- igbt_simple_2/LConn2 -- igbt_simple_1/RConn1

== system interleaved_boost/interleaved_boost_mod1/interleaved_boost/tri-interleaved_boost_pwm/tri-interleaved_legs_modulator ==
  m : Inport  PortDimensions=3
  tri-interleaved_legs_modulator_with_TRGO : Subsystem  mask{f=param.glb_time.fPWM_AFE, m_up=param.boost.pwm.m_up, m_low=param.boost.pwm.m_low, dead_time=param.glb_time.dead_time_AFE, pos_cmd_gate=param.boost.pwm.gate_on, neg_cmd_gate=param.boost.pwm.gate_off, polarity=-1, tc=param.glb_time.tc, double_sampling=param.glb_time.TRGO_AFE_double_update}
      mask prompts: f "Frequency (Hz)"; m_up "Max Input Modulation Value"; m_low "Min Input Modulation Value"; dead_time "Dead Time (s)"; pos_cmd_gate "Positive Gate Voltage (V)"; neg_cmd_gate "Negative Gate Voltage (V)"; polarity "Polarity (pu)"; tc "Sampling time"
  gate_cmds : Outport
  tag scope: TRGO_afe_module_1=global
  wires:
  tri-interleaved_legs_modulator_with_TRGO/1(TRGO) -> [TRGO_afe_module_1]
  m/1 -> tri-interleaved_legs_modulator_with_TRGO/2(m())
  tri-interleaved_legs_modulator_with_TRGO/2(gate_cmds) -> gate_cmds/1
  [time_afe_module_1] -> tri-interleaved_legs_modulator_with_TRGO/1(time_source)

== system interleaved_boost/interleaved_boost_mod1/dcdc_ctrl/boost_control/acquisitions/quantizzation and one step delay 1 ==
  u_in_dcdc_pu : Inport
  quantizzation and one step delay : Subsystem
  u_in_d_dcdc_pu : Outport
  wires:
  u_in_dcdc_pu/1 -> quantizzation and one step delay/1(u_in_dcdc_pu)
  quantizzation and one step delay/1(u_in_d_dcdc_pu) -> u_in_d_dcdc_pu/1

== system interleaved_boost/interleaved_boost_mod1/dcdc_ctrl/boost_control/acquisitions/quantizzation and one step delay 2 ==
  is_abc_dcdc_pu : Inport  PortDimensions=3
  Demux : Demux  Outputs=3
  Mux : Mux  Inputs=3
  quantizzation and one step delay : Subsystem
  is_abc_d_dcdc_pu : Outport
  wires:
  quantizzation and one step delay/2(is_v_d_dcdc_pu) -> Mux/2
  is_abc_dcdc_pu/1 -> Demux/1
  quantizzation and one step delay/3(is_w_d_dcdc_pu) -> Mux/3
  quantizzation and one step delay/1(is_u_d_dcdc_pu) -> Mux/1
  Demux/1 -> quantizzation and one step delay/1(is_u_dcdc_pu)
  Mux/1 -> is_abc_d_dcdc_pu/1
  Demux/3 -> quantizzation and one step delay/3(is_w_dcdc_pu)
  Demux/2 -> quantizzation and one step delay/2(is_v_dcdc_pu)
